simulink subsystem "Final_Project"  (R2024a)
settings: Solver=FixedStepDiscrete  StartTime=0.0  StopTime=10.0  FixedStep=0.001  RelTol=1e-3
undefined symbols (not defined in the file): waypoints
libraries: CarMaker4SL x37, simulink x1
settings Model: Creator=junho.lee  LastModifiedBy=User

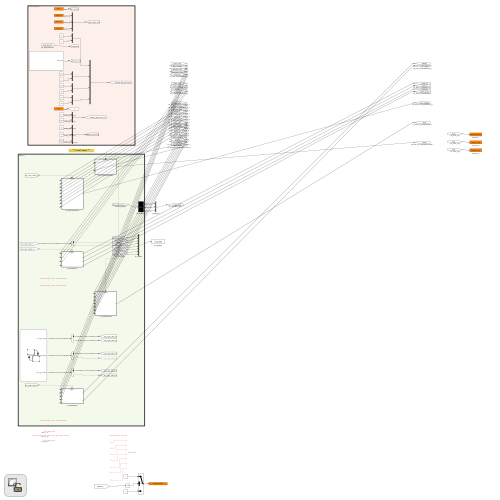
[thumbnail: Simulink's stored preview of the top-level diagram]
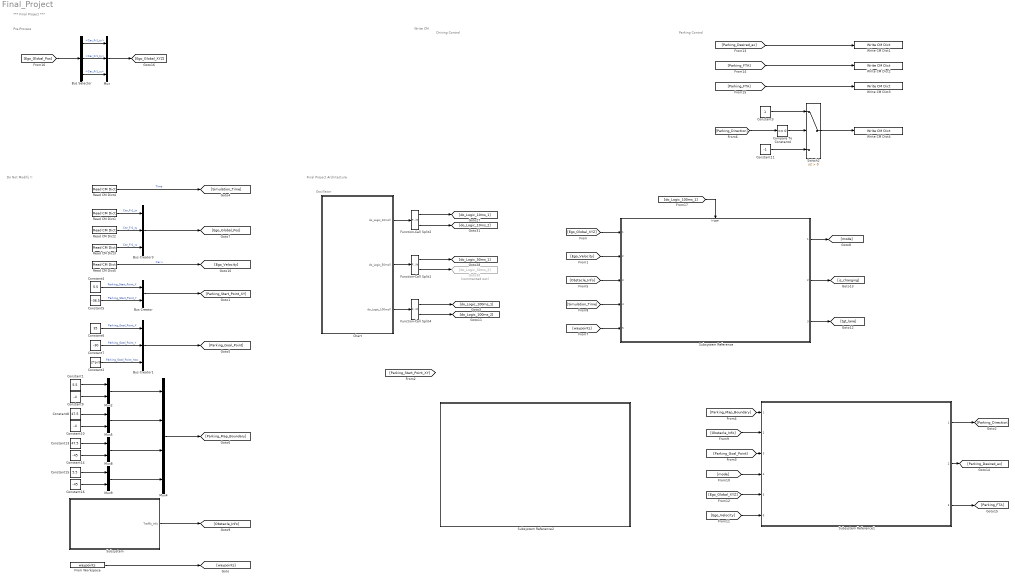
== system Final_Project ==
  note: Do Not Modify !!
  note: *** Final Project ***
  note: Final Project Architecture
  note: Write CM
  note: Oscillator
  note: Parking Control
  note: Driving Control
  note: Pre-Process
  Bus Creator : BusCreator  Inputs=2
  Bus Creator1 : BusCreator  Inputs=3
  Bus Creator3 : BusCreator  Inputs=3
  Bus Selector : BusSelector  OutputSignals=Car_Fr1_tx,Car_Fr1_ty,Car_Fr1_rz
  Chart : Stateflow chart  TreatAsAtomicUnit=on
  Compare To Constant4 : simulink/Logic and Bit Operations/Compare To Constant  relop===  const=0  OutDataTypeStr=boolean
  Constant1 : Constant  Value=5.5
  Constant10 : Constant  Value=-4
  Constant11 : Constant  Value=-1
  Constant13 : Constant  Value=47.5
  Constant14 : Constant  Value=-45
  Constant15 : Constant  Value=5.5
  Constant16 : Constant  Value=-45
  Constant2 : Constant  Value=2*pi/3
  Constant3 : Constant
  Constant4 : Constant  Value=5.5
  Constant5 : Constant  Value=-36.5
  Constant6 : Constant  Value=35
  Constant7 : Constant  Value=-30
  Constant8 : Constant  Value=47.5
  Constant9 : Constant  Value=-4
  From Workspace : Constant  Value=waypoints
  Function-Call Split1 : FunctionCallSplit  IconShape=distinctive  NumOutputPorts=2  OutputPortLayout=default
  Function-Call Split2 : FunctionCallSplit  IconShape=distinctive  NumOutputPorts=2  OutputPortLayout=default
  Function-Call Split4 : FunctionCallSplit  IconShape=distinctive  NumOutputPorts=2  OutputPortLayout=default
  Goto30 : Goto  Commented=on  GotoTag=do_Logic_50ms_2
  Mux : Mux  Inputs=3
  Mux{2,5,8..9} (4 alike) : Mux  Inputs=2
  Mux4 : Mux
  Read CM Dict1 : CarMaker4SL/Read CM Dict  xname=Car.Fr1.tx  xsync=off  xstime=Inherited
  Read CM Dict2 : CarMaker4SL/Read CM Dict  xname=Car.Fr1.ty  xsync=off  xstime=Inherited
  Read CM Dict3 : CarMaker4SL/Read CM Dict  xname=Car.Fr1.rz  xsync=off  xstime=Inherited
  Read CM Dict4 : CarMaker4SL/Read CM Dict  xname=Time  xsync=off  xstime=Inherited
  Read CM Dict5 : CarMaker4SL/Read CM Dict  xname=Car.v  xsync=off  xstime=Inherited
  Subsystem : Subsystem
  Subsystem Reference : Subsystem  ReferencedSubsystem=Supervisor
  Subsystem Reference1 : Subsystem  ReferencedSubsystem=Parking
  Subsystem Reference2 : Subsystem  ReferencedSubsystem=Driving
  Switch2 : Switch  Criteria=u2 > Threshold  SaturateOnIntegerOverflow=off  InputSameDT=off
  Write CM Dict1 : CarMaker4SL/Write CM Dict  xname=AccelCtrl.DesiredAx  xsync=off
  Write CM Dict2 : CarMaker4SL/Write CM Dict  xname=Car.CFR.rz_ext  xsync=off
  Write CM Dict3 : CarMaker4SL/Write CM Dict  xname=Car.CFL.rz_ext  xsync=off
  Write CM Dict4 : CarMaker4SL/Write CM Dict  xname=DM.SelectorCtrl  xsync=off
  wires:
  From Workspace/1 -> [waypoints]
  Constant6/1 -> Bus Creator1/1  "Parking_Goal_Point_X"
  Subsystem/1(Traffic_Info) -> [Obstacle_Info]
  Constant7/1 -> Bus Creator1/2  "Parking_Goal_Point_Y"
  Mux2/1 -> Mux4/1
  Constant2/1 -> Bus Creator1/3  "Parking_Goal_Point_Yaw"
  Mux8/1 -> Mux4/3
  Constant1/1 -> Mux2/1
  Constant9/1 -> Mux2/2
  Constant4/1 -> Bus Creator/1  "Parking_Start_Point_X"
  Read CM Dict5/1 -> [Ego_Velocity]  "Car.v"
  Constant8/1 -> Mux5/1
  Constant10/1 -> Mux5/2
  Constant13/1 -> Mux8/1
  Constant14/1 -> Mux8/2
  Constant15/1 -> Mux9/1
  Constant16/1 -> Mux9/2
  Read CM Dict4/1 -> [Simulation_Time]  "Time"
  Read CM Dict1/1 -> Bus Creator3/1  "Car_Fr1_tx"
  Read CM Dict2/1 -> Bus Creator3/2  "Car_Fr1_ty"
  Function-Call Split2/1 -> [do_Logic_10ms_1]
  Read CM Dict3/1 -> Bus Creator3/3  "Car_Fr1_rz"
  Constant5/1 -> Bus Creator/2  "Parking_Start_Point_Y"
  Bus Creator1/1 -> [Parking_Goal_Point]
  Mux5/1 -> Mux4/2
  Mux9/1 -> Mux4/4
  Bus Creator3/1 -> [Ego_Global_Pos]
  Bus Creator/1 -> [Parking_Start_Point_XY]
  Mux4/1 -> [Parking_Map_Boundary]
  Chart/2(do_Logic_50ms()) -> Function-Call Split1/1
  Function-Call Split1/2 -> Goto30/1
  Chart/1(do_Logic_10ms()) -> Function-Call Split2/1
  Function-Call Split1/1 -> [do_Logic_50ms_1]
  Chart/3(do_Logic_100ms()) -> Function-Call Split4/1
  Function-Call Split2/2 -> [do_Logic_10ms_2]
  Function-Call Split4/1 -> [do_Logic_100ms_1]
  Function-Call Split4/2 -> [do_Logic_100ms_2]
  [Parking_Desired_ax] -> Write CM Dict1/1
  [Parking_FTA] -> Write CM Dict2/1
  [Parking_FTA] -> Write CM Dict3/1
  [Parking_Direction] -> Compare To Constant4/1
  Constant3/1 -> Switch2/1
  Compare To Constant4/1 -> Switch2/2
  Constant11/1 -> Switch2/3
  Switch2/1 -> Write CM Dict4/1
  Subsystem Reference1/1 -> [Parking_Direction]
  [Ego_Global_XYZ] -> Subsystem Reference/1
  [Ego_Velocity] -> Subsystem Reference/2
  [Obstacle_Info] -> Subsystem Reference/3
  [Simulation_Time] -> Subsystem Reference/4
  [waypoints] -> Subsystem Reference/5
  Subsystem Reference/1 -> [mode]
  [Parking_Map_Boundary] -> Subsystem Reference1/1
  [Obstacle_Info] -> Subsystem Reference1/2
  [Parking_Goal_Point] -> Subsystem Reference1/3
  [mode] -> Subsystem Reference1/4
  [Ego_Global_XYZ] -> Subsystem Reference1/5
  [Ego_Velocity] -> Subsystem Reference1/6
  Subsystem Reference1/2 -> [Parking_Desired_ax]
  Subsystem Reference1/3 -> [Parking_FTA]
  [Ego_Global_Pos] -> Bus Selector/1
  Bus Selector/1 -> Mux/1  "<Car_Fr1_tx>"
  Bus Selector/2 -> Mux/2  "<Car_Fr1_ty>"
  Bus Selector/3 -> Mux/3  "<Car_Fr1_rz>"
  Mux/1 -> [Ego_Global_XYZ]
  Subsystem Reference/2 -> [is_changing]
  Subsystem Reference/3 -> [tgt_lane]
  [do_Logic_100ms_1] -> Subsystem Reference/Trigger

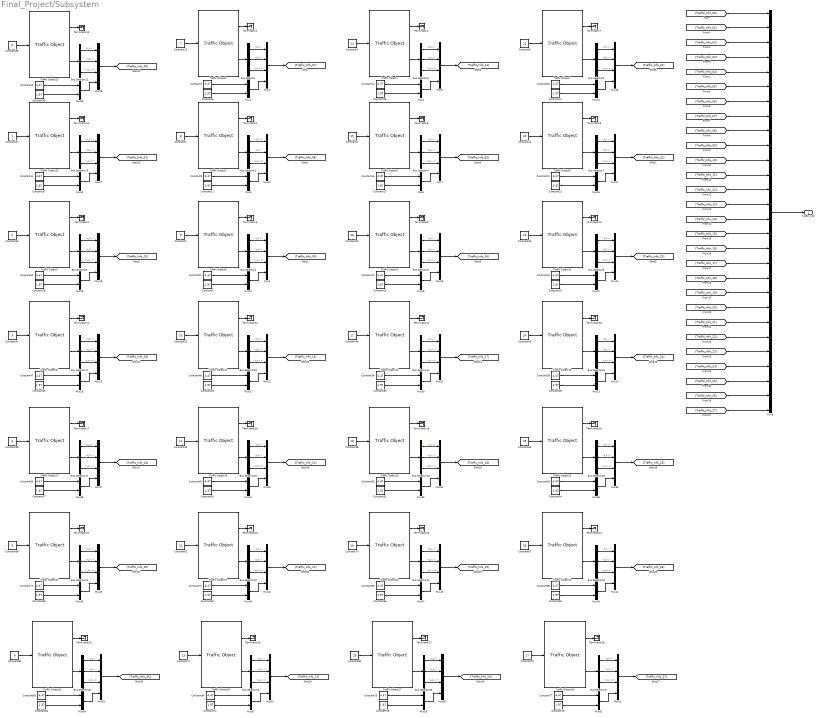
== system Final_Project/Subsystem ==
  Bus Selector{,1..27} (28 alike) : BusSelector  OutputSignals=t_0 x,t_0 y,r_zyx z
  Constant1 : Constant  Value=8
  Constant10 : Constant  Value=7
  Constant{5,8,11,13,15,17,19,21,23,28,33,35,37,39,43,45,50,52,54,57,62,64,66,69,74,76,78,81} (28 alike) : Constant  Value=1.97
  Constant{7,9,12,14,16,18,20,22,30..31,34,38,42,44,47..48,51,53,59..60,63,65,71..72,75,77,83..84} (28 alike) : Constant  Value=4.47
  Constant2 : Constant  Value=9
  Constant24 : Constant  Value=22
  Constant25 : Constant  Value=23
  Constant26 : Constant  Value=2
  Constant27 : Constant
  Constant29 : Constant  Value=16
  Constant3 : Constant  Value=14
  Constant32 : Constant  Value=10
  Constant36 : Constant  Value=0
  Constant4 : Constant  Value=15
  Constant40 : Constant  Value=24
  Constant41 : Constant  Value=3
  Constant46 : Constant  Value=17
  Constant49 : Constant  Value=11
  Constant55 : Constant  Value=25
  Constant56 : Constant  Value=4
  Constant58 : Constant  Value=18
  Constant6 : Constant  Value=21
  Constant61 : Constant  Value=12
  Constant67 : Constant  Value=26
  Constant68 : Constant  Value=5
  Constant70 : Constant  Value=19
  Constant73 : Constant  Value=13
  Constant79 : Constant  Value=27
  Constant80 : Constant  Value=6
  Constant82 : Constant  Value=20
  Mux{1,4,6,8,11,14,16,18..19,21,23,26,28,30,32..33,35,38..39,41,43,46..47,49,51,54..55,57} (28 alike) : Mux  Inputs=2
  Mux{2..3,5,7,10,12..13,15,17,20,22,24..25,27,29,31,34,36..37,40,42,44..45,48,50,52..53,56} (28 alike) : Mux
  Mux9 : Mux  Inputs=28
  Terminator{1..28} (28 alike) : Terminator
  Traffic Object1 : CarMaker4SL/Traffic Object  xname=T07  ximode=Traffic Id  xstime=Inherited
      settings: SourceProductName=CarMaker4SL
  Traffic Object10 : CarMaker4SL/Traffic Object  xname=T23  ximode=Traffic Id  xstime=Inherited
      settings: SourceProductName=CarMaker4SL
  Traffic Object11 : CarMaker4SL/Traffic Object  xname=T03  ximode=Traffic Id  xstime=Inherited
      settings: SourceProductName=CarMaker4SL
  Traffic Object12 : CarMaker4SL/Traffic Object  xname=T10  ximode=Traffic Id  xstime=Inherited
      settings: SourceProductName=CarMaker4SL
  Traffic Object13 : CarMaker4SL/Traffic Object  xname=T00  ximode=Traffic Id  xstime=Inherited
      settings: SourceProductName=CarMaker4SL
  Traffic Object14 : CarMaker4SL/Traffic Object  xname=T17  ximode=Traffic Id  xstime=Inherited
      settings: SourceProductName=CarMaker4SL
  Traffic Object15 : CarMaker4SL/Traffic Object  xname=T01  ximode=Traffic Id  xstime=Inherited
      settings: SourceProductName=CarMaker4SL
  Traffic Object16 : CarMaker4SL/Traffic Object  xname=T24  ximode=Traffic Id  xstime=Inherited
      settings: SourceProductName=CarMaker4SL
  Traffic Object17 : CarMaker4SL/Traffic Object  xname=T04  ximode=Traffic Id  xstime=Inherited
      settings: SourceProductName=CarMaker4SL
  Traffic Object18 : CarMaker4SL/Traffic Object  xname=T11  ximode=Traffic Id  xstime=Inherited
      settings: SourceProductName=CarMaker4SL
  Traffic Object19 : CarMaker4SL/Traffic Object  xname=T18  ximode=Traffic Id  xstime=Inherited
      settings: SourceProductName=CarMaker4SL
  Traffic Object2 : CarMaker4SL/Traffic Object  xname=T08  ximode=Traffic Id  xstime=Inherited
      settings: SourceProductName=CarMaker4SL
  Traffic Object20 : CarMaker4SL/Traffic Object  xname=T25  ximode=Traffic Id  xstime=Inherited
      settings: SourceProductName=CarMaker4SL
  Traffic Object21 : CarMaker4SL/Traffic Object  xname=T05  ximode=Traffic Id  xstime=Inherited
      settings: SourceProductName=CarMaker4SL
  Traffic Object22 : CarMaker4SL/Traffic Object  xname=T12  ximode=Traffic Id  xstime=Inherited
      settings: SourceProductName=CarMaker4SL
  Traffic Object23 : CarMaker4SL/Traffic Object  xname=T19  ximode=Traffic Id  xstime=Inherited
      settings: SourceProductName=CarMaker4SL
  Traffic Object24 : CarMaker4SL/Traffic Object  xname=T26  ximode=Traffic Id  xstime=Inherited
      settings: SourceProductName=CarMaker4SL
  Traffic Object25 : CarMaker4SL/Traffic Object  xname=T06  ximode=Traffic Id  xstime=Inherited
      settings: SourceProductName=CarMaker4SL
  Traffic Object26 : CarMaker4SL/Traffic Object  xname=T13  ximode=Traffic Id  xstime=Inherited
      settings: SourceProductName=CarMaker4SL
  Traffic Object27 : CarMaker4SL/Traffic Object  xname=T20  ximode=Traffic Id  xstime=Inherited
      settings: SourceProductName=CarMaker4SL
  Traffic Object28 : CarMaker4SL/Traffic Object  xname=T27  ximode=Traffic Id  xstime=Inherited
      settings: SourceProductName=CarMaker4SL
  Traffic Object3 : CarMaker4SL/Traffic Object  xname=T02  ximode=Traffic Id  xstime=Inherited
      settings: SourceProductName=CarMaker4SL
  Traffic Object4 : CarMaker4SL/Traffic Object  xname=T14  ximode=Traffic Id  xstime=Inherited
      settings: SourceProductName=CarMaker4SL
  Traffic Object5 : CarMaker4SL/Traffic Object  xname=T15  ximode=Traffic Id  xstime=Inherited
      settings: SourceProductName=CarMaker4SL
  Traffic Object6 : CarMaker4SL/Traffic Object  xname=T09  ximode=Traffic Id  xstime=Inherited
      settings: SourceProductName=CarMaker4SL
  Traffic Object7 : CarMaker4SL/Traffic Object  xname=T21  ximode=Traffic Id  xstime=Inherited
      settings: SourceProductName=CarMaker4SL
  Traffic Object8 : CarMaker4SL/Traffic Object  xname=T22  ximode=Traffic Id  xstime=Inherited
      settings: SourceProductName=CarMaker4SL
  Traffic Object9 : CarMaker4SL/Traffic Object  xname=T16  ximode=Traffic Id  xstime=Inherited
      settings: SourceProductName=CarMaker4SL
  Traffic_Info : Outport
  wires:
  [Traffic_Info_21] -> Mux9/22
  [Traffic_Info_27] -> Mux9/28
  [Traffic_Info_26] -> Mux9/27
  [Traffic_Info_22] -> Mux9/23
  [Traffic_Info_25] -> Mux9/26
  [Traffic_Info_24] -> Mux9/25
  [Traffic_Info_23] -> Mux9/24
  [Traffic_Info_14] -> Mux9/15
  [Traffic_Info_20] -> Mux9/21
  [Traffic_Info_19] -> Mux9/20
  [Traffic_Info_15] -> Mux9/16
  [Traffic_Info_18] -> Mux9/19
  [Traffic_Info_17] -> Mux9/18
  [Traffic_Info_16] -> Mux9/17
  [Traffic_Info_07] -> Mux9/8
  [Traffic_Info_13] -> Mux9/14
  [Traffic_Info_12] -> Mux9/13
  [Traffic_Info_08] -> Mux9/9
  [Traffic_Info_11] -> Mux9/12
  [Traffic_Info_10] -> Mux9/11
  [Traffic_Info_09] -> Mux9/10
  Constant84/1 -> Mux57/1
  Traffic Object27/2 -> Bus Selector26/1
  Constant83/1 -> Mux54/1
  Mux54/1 -> Mux53/4
  Bus Selector25/1 -> Mux53/1  "<t_0 x>"
  Bus Selector26/2 -> Mux56/2  "<t_0 y>"
  Mux56/1 -> [Traffic_Info_20]
  Constant73/1 -> Traffic Object26/1
  Bus Selector25/3 -> Mux53/3  "<r_zyx z>"
  Constant82/1 -> Traffic Object27/1
  Mux53/1 -> [Traffic_Info_06]
  Traffic Object28/1 -> Terminator28/1
  Traffic Object25/1 -> Terminator25/1
  Traffic Object25/2 -> Bus Selector25/1
  Constant81/1 -> Mux54/2
  Bus Selector24/3 -> Mux50/3  "<r_zyx z>"
  Traffic Object26/1 -> Terminator26/1
  Bus Selector24/1 -> Mux50/1  "<t_0 x>"
  Traffic Object27/1 -> Terminator27/1
  Traffic Object26/2 -> Bus Selector24/1
  Mux57/1 -> Mux50/4
  Bus Selector26/1 -> Mux56/1  "<t_0 x>"
  Constant76/1 -> Mux55/2
  Bus Selector24/2 -> Mux50/2  "<t_0 y>"
  Bus Selector27/2 -> Mux52/2  "<t_0 y>"
  Mux50/1 -> [Traffic_Info_13]
  Bus Selector25/2 -> Mux53/2  "<t_0 y>"
  Constant80/1 -> Traffic Object25/1
  Constant75/1 -> Mux55/1
  Bus Selector26/3 -> Mux56/3  "<r_zyx z>"
  Mux55/1 -> Mux56/4
  Constant74/1 -> Mux57/2
  Mux51/1 -> Mux52/4
  Bus Selector27/3 -> Mux52/3  "<r_zyx z>"
  Constant77/1 -> Mux51/1
  Traffic Object28/2 -> Bus Selector27/1
  Constant78/1 -> Mux51/2
  Bus Selector27/1 -> Mux52/1  "<t_0 x>"
  Mux52/1 -> [Traffic_Info_27]
  Constant79/1 -> Traffic Object28/1
  Constant72/1 -> Mux49/1
  Traffic Object23/2 -> Bus Selector22/1
  Constant71/1 -> Mux46/1
  Mux46/1 -> Mux45/4
  Bus Selector21/1 -> Mux45/1  "<t_0 x>"
  Bus Selector22/2 -> Mux48/2  "<t_0 y>"
  Mux48/1 -> [Traffic_Info_19]
  Constant61/1 -> Traffic Object22/1
  Bus Selector21/3 -> Mux45/3  "<r_zyx z>"
  Constant70/1 -> Traffic Object23/1
  Mux45/1 -> [Traffic_Info_05]
  Traffic Object24/1 -> Terminator24/1
  Traffic Object21/1 -> Terminator21/1
  Traffic Object21/2 -> Bus Selector21/1
  Constant69/1 -> Mux46/2
  Bus Selector20/3 -> Mux42/3  "<r_zyx z>"
  Traffic Object22/1 -> Terminator22/1
  Bus Selector20/1 -> Mux42/1  "<t_0 x>"
  Traffic Object23/1 -> Terminator23/1
  Traffic Object22/2 -> Bus Selector20/1
  Mux49/1 -> Mux42/4
  Bus Selector22/1 -> Mux48/1  "<t_0 x>"
  Constant64/1 -> Mux47/2
  Bus Selector20/2 -> Mux42/2  "<t_0 y>"
  Bus Selector23/2 -> Mux44/2  "<t_0 y>"
  Mux42/1 -> [Traffic_Info_12]
  Bus Selector21/2 -> Mux45/2  "<t_0 y>"
  Constant68/1 -> Traffic Object21/1
  Constant63/1 -> Mux47/1
  Bus Selector22/3 -> Mux48/3  "<r_zyx z>"
  Mux47/1 -> Mux48/4
  Constant62/1 -> Mux49/2
  Mux43/1 -> Mux44/4
  Bus Selector23/3 -> Mux44/3  "<r_zyx z>"
  Constant65/1 -> Mux43/1
  Traffic Object24/2 -> Bus Selector23/1
  Constant66/1 -> Mux43/2
  Bus Selector23/1 -> Mux44/1  "<t_0 x>"
  Mux44/1 -> [Traffic_Info_26]
  Constant67/1 -> Traffic Object24/1
  Constant60/1 -> Mux41/1
  Traffic Object19/2 -> Bus Selector18/1
  Constant59/1 -> Mux38/1
  Mux38/1 -> Mux37/4
  Bus Selector17/1 -> Mux37/1  "<t_0 x>"
  Bus Selector18/2 -> Mux40/2  "<t_0 y>"
  Mux40/1 -> [Traffic_Info_18]
  Constant49/1 -> Traffic Object18/1
  Bus Selector17/3 -> Mux37/3  "<r_zyx z>"
  Constant58/1 -> Traffic Object19/1
  Mux37/1 -> [Traffic_Info_04]
  Traffic Object20/1 -> Terminator20/1
  Traffic Object17/1 -> Terminator17/1
  Traffic Object17/2 -> Bus Selector17/1
  Constant57/1 -> Mux38/2
  Bus Selector16/3 -> Mux34/3  "<r_zyx z>"
  Traffic Object18/1 -> Terminator18/1
  Bus Selector16/1 -> Mux34/1  "<t_0 x>"
  Traffic Object19/1 -> Terminator19/1
  Traffic Object18/2 -> Bus Selector16/1
  Mux41/1 -> Mux34/4
  Bus Selector18/1 -> Mux40/1  "<t_0 x>"
  Constant52/1 -> Mux39/2
  Bus Selector16/2 -> Mux34/2  "<t_0 y>"
  Bus Selector19/2 -> Mux36/2  "<t_0 y>"
  Mux34/1 -> [Traffic_Info_11]
  Bus Selector17/2 -> Mux37/2  "<t_0 y>"
  Constant56/1 -> Traffic Object17/1
  Constant51/1 -> Mux39/1
  Bus Selector18/3 -> Mux40/3  "<r_zyx z>"
  Mux39/1 -> Mux40/4
  Constant50/1 -> Mux41/2
  Mux35/1 -> Mux36/4
  Bus Selector19/3 -> Mux36/3  "<r_zyx z>"
  Constant53/1 -> Mux35/1
  Traffic Object20/2 -> Bus Selector19/1
  Constant54/1 -> Mux35/2
  Bus Selector19/1 -> Mux36/1  "<t_0 x>"
  Mux36/1 -> [Traffic_Info_25]
  Constant55/1 -> Traffic Object20/1
  Constant48/1 -> Mux32/1
  Traffic Object14/2 -> Bus Selector14/1
  Constant47/1 -> Mux28/1
  Mux28/1 -> Mux25/4
  Bus Selector11/1 -> Mux25/1  "<t_0 x>"
  Bus Selector14/2 -> Mux31/2  "<t_0 y>"
  Mux31/1 -> [Traffic_Info_17]
  Constant32/1 -> Traffic Object12/1
  Bus Selector11/3 -> Mux25/3  "<r_zyx z>"
  Constant46/1 -> Traffic Object14/1
  Mux25/1 -> [Traffic_Info_03]
  Traffic Object16/1 -> Terminator16/1
  Traffic Object11/1 -> Terminator11/1
  Traffic Object11/2 -> Bus Selector11/1
  Constant45/1 -> Mux28/2
  Bus Selector10/3 -> Mux22/3  "<r_zyx z>"
  Traffic Object12/1 -> Terminator12/1
  Bus Selector10/1 -> Mux22/1  "<t_0 x>"
  Traffic Object14/1 -> Terminator14/1
  Traffic Object12/2 -> Bus Selector10/1
  Mux32/1 -> Mux22/4
  Bus Selector14/1 -> Mux31/1  "<t_0 x>"
  Constant35/1 -> Mux30/2
  Bus Selector10/2 -> Mux22/2  "<t_0 y>"
  Bus Selector15/2 -> Mux24/2  "<t_0 y>"
  Mux22/1 -> [Traffic_Info_10]
  Bus Selector11/2 -> Mux25/2  "<t_0 y>"
  Constant41/1 -> Traffic Object11/1
  Constant34/1 -> Mux30/1
  Bus Selector14/3 -> Mux31/3  "<r_zyx z>"
  Mux30/1 -> Mux31/4
  Constant33/1 -> Mux32/2
  Mux23/1 -> Mux24/4
  Bus Selector15/3 -> Mux24/3  "<r_zyx z>"
  Constant38/1 -> Mux23/1
  Traffic Object16/2 -> Bus Selector15/1
  Constant39/1 -> Mux23/2
  Bus Selector15/1 -> Mux24/1  "<t_0 x>"
  Mux24/1 -> [Traffic_Info_24]
  Constant40/1 -> Traffic Object16/1
  Constant31/1 -> Mux21/1
  Traffic Object9/2 -> Bus Selector8/1
  Constant30/1 -> Mux18/1
  Mux18/1 -> Mux13/4
  Bus Selector5/1 -> Mux13/1  "<t_0 x>"
  Bus Selector8/2 -> Mux20/2  "<t_0 y>"
  Mux20/1 -> [Traffic_Info_16]
  Constant2/1 -> Traffic Object6/1
  Bus Selector5/3 -> Mux13/3  "<r_zyx z>"
  Constant29/1 -> Traffic Object9/1
  Mux13/1 -> [Traffic_Info_02]
  Traffic Object10/1 -> Terminator10/1
  Traffic Object3/1 -> Terminator3/1
  Traffic Object3/2 -> Bus Selector5/1
  Constant28/1 -> Mux18/2
  Bus Selector2/3 -> Mux3/3  "<r_zyx z>"
  Traffic Object6/1 -> Terminator6/1
  Bus Selector2/1 -> Mux3/1  "<t_0 x>"
  Traffic Object9/1 -> Terminator9/1
  Traffic Object6/2 -> Bus Selector2/1
  Mux21/1 -> Mux3/4
  Bus Selector8/1 -> Mux20/1  "<t_0 x>"
  Constant13/1 -> Mux19/2
  Bus Selector2/2 -> Mux3/2  "<t_0 y>"
  Bus Selector9/2 -> Mux12/2  "<t_0 y>"
  Mux3/1 -> [Traffic_Info_09]
  Bus Selector5/2 -> Mux13/2  "<t_0 y>"
  Constant26/1 -> Traffic Object3/1
  Constant12/1 -> Mux19/1
  Bus Selector8/3 -> Mux20/3  "<r_zyx z>"
  Mux19/1 -> Mux20/4
  Constant5/1 -> Mux21/2
  Mux11/1 -> Mux12/4
  Bus Selector9/3 -> Mux12/3  "<r_zyx z>"
  Constant18/1 -> Mux11/1
  Traffic Object10/2 -> Bus Selector9/1
  Constant19/1 -> Mux11/2
  Bus Selector9/1 -> Mux12/1  "<t_0 x>"
  Mux12/1 -> [Traffic_Info_23]
  Constant25/1 -> Traffic Object10/1
  Constant27/1 -> Traffic Object15/1
  Bus Selector12/3 -> Mux29/3  "<r_zyx z>"
  Mux29/1 -> [Traffic_Info_00]
  Constant43/1 -> Mux26/2
  Bus Selector13/2 -> Mux27/2  "<t_0 y>"
  Bus Selector13/3 -> Mux27/3  "<r_zyx z>"
  Mux33/1 -> Mux27/4
  Bus Selector13/1 -> Mux27/1  "<t_0 x>"
  Constant44/1 -> Mux33/1
  Bus Selector12/2 -> Mux29/2  "<t_0 y>"
  Traffic Object15/1 -> Terminator15/1
  Traffic Object13/1 -> Terminator13/1
  Traffic Object15/2 -> Bus Selector13/1
  Mux27/1 -> [Traffic_Info_01]
  Constant42/1 -> Mux26/1
  Constant36/1 -> Traffic Object13/1
  Bus Selector12/1 -> Mux29/1  "<t_0 x>"
  Mux26/1 -> Mux29/4
  Traffic Object13/2 -> Bus Selector12/1
  Constant37/1 -> Mux33/2
  Constant24/1 -> Traffic Object8/1
  Traffic Object8/1 -> Terminator8/1
  Bus Selector7/2 -> Mux17/2  "<t_0 y>"
  Mux17/1 -> [Traffic_Info_22]
  Bus Selector7/1 -> Mux17/1  "<t_0 x>"
  Bus Selector7/3 -> Mux17/3  "<r_zyx z>"
  Traffic Object8/2 -> Bus Selector7/1
  Constant23/1 -> Mux16/2
  Constant22/1 -> Mux16/1
  Mux16/1 -> Mux17/4
  Mux14/1 -> Mux15/4
  Constant20/1 -> Mux14/1
  Constant21/1 -> Mux14/2
  Mux6/1 -> Mux7/4
  Constant16/1 -> Mux6/1
  Constant17/1 -> Mux6/2
  Mux4/1 -> Mux5/4
  Constant14/1 -> Mux4/1
  Constant15/1 -> Mux4/2
  Mux8/1 -> Mux10/4
  Constant9/1 -> Mux8/1
  Constant11/1 -> Mux8/2
  Constant7/1 -> Mux1/1
  Mux1/1 -> Mux2/4
  Constant8/1 -> Mux1/2
  [Traffic_Info_03] -> Mux9/4
  [Traffic_Info_04] -> Mux9/5
  [Traffic_Info_05] -> Mux9/6
  [Traffic_Info_06] -> Mux9/7
  [Traffic_Info_02] -> Mux9/3
  Mux9/1 -> Traffic_Info/1
  [Traffic_Info_01] -> Mux9/2
  [Traffic_Info_00] -> Mux9/1
  Mux2/1 -> [Traffic_Info_07]
  Traffic Object7/2 -> Bus Selector6/1
  Bus Selector6/3 -> Mux15/3  "<r_zyx z>"
  Bus Selector6/1 -> Mux15/1  "<t_0 x>"
  Mux15/1 -> [Traffic_Info_21]
  Bus Selector6/2 -> Mux15/2  "<t_0 y>"
  Traffic Object5/2 -> Bus Selector4/1
  Bus Selector4/3 -> Mux7/3  "<r_zyx z>"
  Bus Selector4/1 -> Mux7/1  "<t_0 x>"
  Mux7/1 -> [Traffic_Info_15]
  Bus Selector4/2 -> Mux7/2  "<t_0 y>"
  Traffic Object4/2 -> Bus Selector3/1
  Bus Selector3/3 -> Mux5/3  "<r_zyx z>"
  Bus Selector3/1 -> Mux5/1  "<t_0 x>"
  Mux5/1 -> [Traffic_Info_14]
  Bus Selector3/2 -> Mux5/2  "<t_0 y>"
  Traffic Object2/2 -> Bus Selector1/1
  Bus Selector1/3 -> Mux10/3  "<r_zyx z>"
  Bus Selector1/1 -> Mux10/1  "<t_0 x>"
  Mux10/1 -> [Traffic_Info_08]
  Bus Selector1/2 -> Mux10/2  "<t_0 y>"
  Bus Selector/3 -> Mux2/3  "<r_zyx z>"
  Bus Selector/2 -> Mux2/2  "<t_0 y>"
  Bus Selector/1 -> Mux2/1  "<t_0 x>"
  Traffic Object1/2 -> Bus Selector/1
  Traffic Object7/1 -> Terminator7/1
  Constant6/1 -> Traffic Object7/1
  Traffic Object5/1 -> Terminator5/1
  Constant4/1 -> Traffic Object5/1
  Constant3/1 -> Traffic Object4/1
  Traffic Object4/1 -> Terminator4/1
  Constant1/1 -> Traffic Object2/1
  Traffic Object2/1 -> Terminator2/1
  Traffic Object1/1 -> Terminator1/1
  Constant10/1 -> Traffic Object1/1

== stateflow chart Final_Project/Chart ==
  (default) -> (junction 1)
  (junction 1) -> (junction 3) [order 1] : [mod(i,10) == 0]
      | {do_Logic_10ms;}
  (junction 1) -> (junction 7) [order 2]
  (junction 3) -> (junction 5)
  (junction 5) -> (junction 7)
  (junction 7) -> (junction 10)
  (junction 10) -> (junction 12) [order 1] : [mod(i, 50) == 0]
      | {do_Logic_50ms;}
  (junction 10) -> (junction 18) [order 2]
  (junction 12) -> (junction 16)
  (junction 16) -> (junction 18)
  (junction 18) -> (junction 25)
  (junction 25) -> (junction 27) [order 1] : [mod(i,100) == 0]
      | {do_Logic_100ms;}
  (junction 25) -> (junction 21) [order 2]
  (junction 27) -> (junction 29) : {i = 0;}
  (junction 29) -> (junction 21)
  (junction 21) -> (junction 32) : {i = i +1;}
  data: i local =0
  events: do_Logic_10ms output FUNCTION_CALL_EVENT; do_Logic_50ms output FUNCTION_CALL_EVENT; do_Logic_100ms output FUNCTION_CALL_EVENT
